simulink model "ps_25V_12kA_r"  (R2026b)
settings: Solver=ode23tb  StopTime=param.sim.simlength  FixedStep=param.glb_time.tc  MaxStep=param.glb_time.tc
values from neighbouring files (symbols this model uses):
  param = struct()    [init_model.m]
undefined symbols (not defined in the file or in its folder): magnitude
libraries: fl_lib x106, nesl_utility x71, afe_uvw_ctrl x5, ee_legacy_lib x5, discrete_time_low_pass_filter x2, three_windings_transformer x2, pi_ctrl x2, threephase_inductor_lib x1, dclink_for_two_levels x1, three_phase_pwm_modulator x1, three_phase_inverter_ideal_switch_based_model x1, three_phase_inverter_igbt_advanced_thermal_model x1
(part 1 of 5)
settings Model: Creator=dbagn  LastModifiedBy=d.bagnara
settings SolverCC: SolverResetMethod=Robust  ZeroCrossControl=DisableAll
settings DataIOCC: DSMLogging=off  ReturnWorkspaceOutputs=off  SaveOutput=off  SaveTime=off  SignalLogging=off
settings OptimizationCC: ReuseModelBlockBuffer=off
settings SFSimCC: CustomCodeUndefinedFunction=ThrowError  DefaultCustomCodeDeterministicFunctions=All
settings SFSimCC: SimCustomHeaderCode=|
  | #include "rpi.h"
  | #include "mavgflt.h"
  | #include "mavgflt_simulink.h"
  | #include "mavgflts.h"
  | #include "mavgflts_simulink.h"
  | #include "dsmavgflt.h"
  | #include "dsmavgflt_simulink.h"
  | #include "bemf_obsv.h"
  | #include "bemf_obsv_simulink.h"
  | #include "bemf_obsv_load_est.h"
  | #include "bemf_obsv_load_est_simulink.h"
  | #include "dqvector_pi.h"
  | #include "dqvector_pi_simulink.h"
  | #include "sv_pwm_simulink.h"
  | #include "sv_pwm.h"
  | #include "sv_pwm_cm_simulink.h"
  | #include "sv_pwm_cm.h"
  | #include "first_harmonic_tracker.h"
  | #include "first_harmonic_tracker_simulink.h"
  | #include "dqpll_thyr.h"
  | #include "dqpll_thyr_simulink.h"
  | #include "dqpll_grid.h"
  | #include "dqpll_grid_simulink.h"
  | #include "linear_double_integrator_observer_simulink.h"
  | #include "linear_double_integrator_observer.h"
settings SFSimCC: SimUserIncludeDirs=|
  | include
  | src
settings SFSimCC: SimUserSources=|
  | "rpi.c"
  | "mavgflt_simulink.c"
  | "mavgflt.c"
  | "mavgflts_simulink.c"
  | "mavgflts.c"
  | "dsmavgflt_simulink.c"
  | "dsmavgflt.c"
  | "bemf_obsv_simulink.c"
  | "bemf_obsv.c"
  | "bemf_obsv_load_est_simulink.c"
  | "bemf_obsv_load_est.c"
  | "dqvector_pi.c"
  | "dqvector_pi_simulink.c"
  | "sv_pwm_simulink.c"
  | "sv_pwm.c"
  | "sv_pwm_cm_simulink.c"
  | "sv_pwm_cm.c"
  | "first_harmonic_tracker_simulink.c"
  | "first_harmonic_tracker.c"
  | "dqpll_thyr_simulink.c"
  | "dqpll_thyr.c"
  | "dqpll_grid_simulink.c"
  | "dqpll_grid.c"
  | "linear_double_integrator_observer_simulink.c"
  | "linear_double_integrator_observer.c"
settings RTWCC: DLArmComputeVersion=19.05
settings SimscapeCC: SimscapeUseEnergyAccounting=off

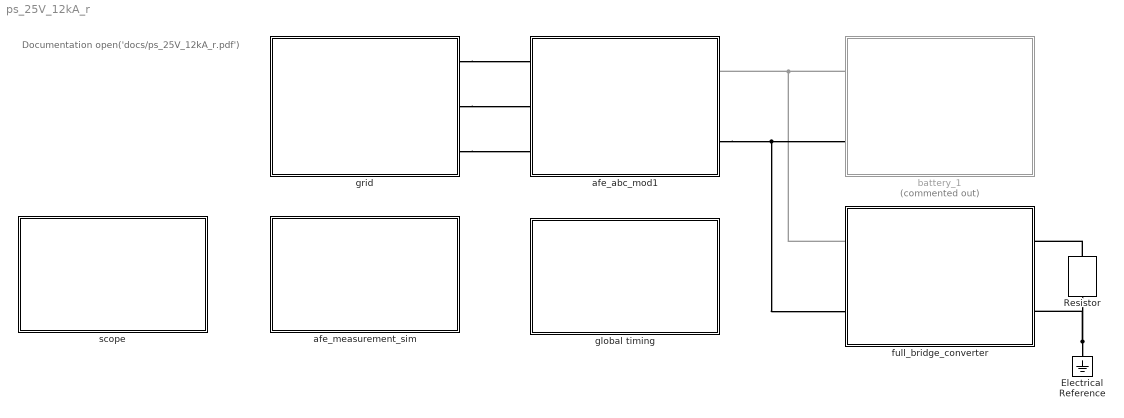
== system ps_25V_12kA_r ==
  note: Documentation
      | open('docs/ps_25V_12kA_r.pdf')
  Electrical Reference : fl_lib/Electrical/Electrical Elements/Electrical Reference
  Resistor : fl_lib/Electrical/Electrical Elements/Resistor  R=param.load.R Ohm  i_specify=off  i_priority=None  i=0 A  i_nominal_specify=off  i_nominal_value=1  i_nominal_unit=A  v_specify=off  v_priority=None  v=0 V  v_nominal_specify=off  v_nominal_value=1  v_nominal_unit=V
  afe_abc_mod1 : Subsystem
  afe_measurement_sim : Subsystem
  battery_1 : Subsystem  Commented=on
  full_bridge_converter : Subsystem
  global timing : Subsystem
  grid : Subsystem
  scope : Subsystem
  connections:
  grid/RConn1 -- afe_abc_mod1/LConn1
  grid/RConn3 -- afe_abc_mod1/LConn3
  grid/RConn2 -- afe_abc_mod1/LConn2
  battery_1/RConn1 -- full_bridge_converter/LConn1 -- afe_abc_mod1/RConn1
  afe_abc_mod1/RConn2 -- full_bridge_converter/LConn2 -- battery_1/RConn2
  Electrical Reference/LConn1 -- Resistor/RConn1 -- full_bridge_converter/RConn2
  Resistor/LConn1 -- full_bridge_converter/RConn1

== system ps_25V_12kA_r/afe_abc_mod1 ==
  AFE_control : Subsystem
  LCL_filter : Subsystem
  afe : Subsystem
  brake : Subsystem
  ug_a : PMIOPort  Side=Left
  Udc(+) : PMIOPort  Port=2  Side=Right
  ug_b : PMIOPort  Port=3  Side=Left
  Udc(-) : PMIOPort  Port=4  Side=Right
  ug_c : PMIOPort  Port=5  Side=Left
  wires:
  AFE_control/1(dabc_out) -> afe/1(dabc)
  connections:
  Udc(-)/RConn1 -- brake/LConn2 -- afe/RConn2
  Udc(+)/RConn1 -- brake/LConn1 -- afe/RConn1
  LCL_filter/LConn1 -- afe/LConn1
  LCL_filter/LConn2 -- afe/LConn2
  LCL_filter/LConn3 -- afe/LConn3
  ug_a/RConn1 -- LCL_filter/RConn1
  ug_b/RConn1 -- LCL_filter/RConn2
  ug_c/RConn1 -- LCL_filter/RConn3

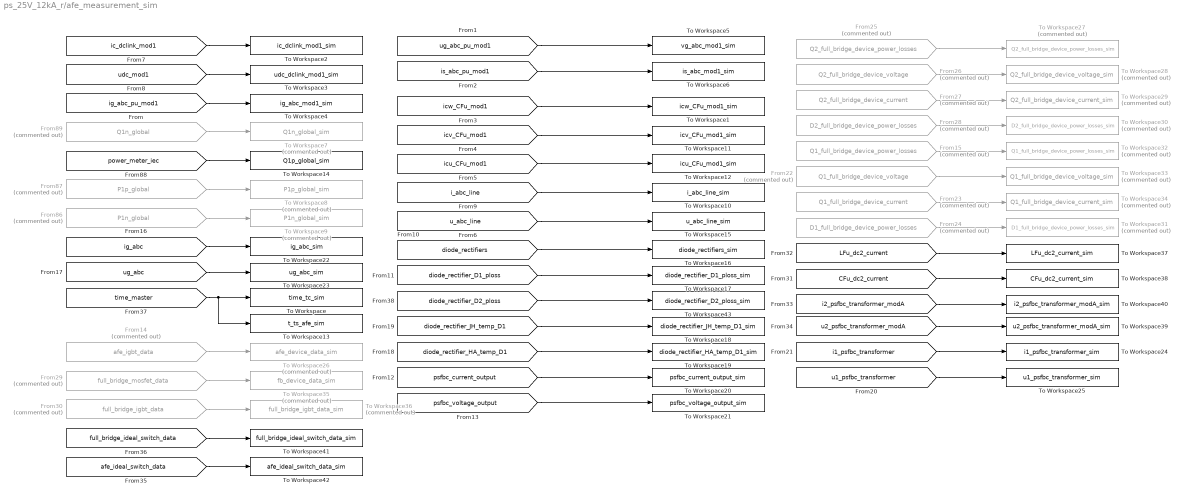
== system ps_25V_12kA_r/afe_measurement_sim ==
  From14 : From  Commented=on  GotoTag=afe_igbt_data
  From15 : From  Commented=on  GotoTag=Q1_full_bridge_device_power_losses
  From22 : From  Commented=on  GotoTag=Q1_full_bridge_device_voltage
  From23 : From  Commented=on  GotoTag=Q1_full_bridge_device_current
  From24 : From  Commented=on  GotoTag=D1_full_bridge_device_power_losses
  From25 : From  Commented=on  GotoTag=Q2_full_bridge_device_power_losses
  From26 : From  Commented=on  GotoTag=Q2_full_bridge_device_voltage
  From27 : From  Commented=on  GotoTag=Q2_full_bridge_device_current
  From28 : From  Commented=on  GotoTag=D2_full_bridge_device_power_losses
  From29 : From  Commented=on  GotoTag=full_bridge_mosfet_data
  From30 : From  Commented=on  GotoTag=full_bridge_igbt_data
  From86 : From  Commented=on  GotoTag=P1n_global
  From87 : From  Commented=on  GotoTag=P1p_global
  From89 : From  Commented=on  GotoTag=Q1n_global
  To Workspace : ToWorkspace  VariableName=time_tc_sim  SampleTime=param.glb_time.tc
      settings: MaxDataPoints=param.glb_time.Nc  Decimation=param.glb_time.decimation_tc
  To Workspace1 : ToWorkspace  VariableName=icw_CFu_mod1_sim  SampleTime=param.glb_time.tc
      settings: MaxDataPoints=param.glb_time.Nc  Decimation=param.glb_time.decimation_tc
  To Workspace10 : ToWorkspace  VariableName=i_abc_line_sim  SampleTime=param.glb_time.tc
      settings: MaxDataPoints=param.glb_time.Nc  Decimation=param.glb_time.decimation_tc
  To Workspace11 : ToWorkspace  VariableName=icv_CFu_mod1_sim  SampleTime=param.glb_time.tc
      settings: MaxDataPoints=param.glb_time.Nc  Decimation=param.glb_time.decimation_tc
  To Workspace12 : ToWorkspace  VariableName=icu_CFu_mod1_sim  SampleTime=param.glb_time.tc
      settings: MaxDataPoints=param.glb_time.Nc  Decimation=param.glb_time.decimation_tc
  To Workspace13 : ToWorkspace  VariableName=t_ts_afe_sim  SampleTime=param.glb_time.ts_afe
      settings: MaxDataPoints=param.glb_time.Ns_afe
  To Workspace14 : ToWorkspace  VariableName=Q1p_global_sim  SampleTime=param.glb_time.tc
      settings: MaxDataPoints=param.glb_time.Nc  Decimation=param.glb_time.decimation_tc
  To Workspace15 : ToWorkspace  VariableName=u_abc_line_sim  SampleTime=param.glb_time.tc
      settings: MaxDataPoints=param.glb_time.Nc  Decimation=param.glb_time.decimation_tc
  To Workspace16 : ToWorkspace  VariableName=diode_rectifiers_sim  SampleTime=param.glb_time.tc
      settings: MaxDataPoints=param.glb_time.Nc  Decimation=param.glb_time.decimation_tc
  To Workspace17 : ToWorkspace  VariableName=diode_rectifier_D1_ploss_sim  SampleTime=param.glb_time.tc
      settings: MaxDataPoints=param.glb_time.Nc  Decimation=param.glb_time.decimation_tc
  To Workspace18 : ToWorkspace  VariableName=diode_rectifier_JH_temp_D1_sim  SampleTime=param.glb_time.tc
      settings: MaxDataPoints=param.glb_time.Nc  Decimation=param.glb_time.decimation_tc
  To Workspace19 : ToWorkspace  VariableName=diode_rectifier_HA_temp_D1_sim  SampleTime=param.glb_time.tc
      settings: MaxDataPoints=param.glb_time.Nc  Decimation=param.glb_time.decimation_tc
  To Workspace2 : ToWorkspace  VariableName=ic_dclink_mod1_sim  SampleTime=param.glb_time.tc
      settings: MaxDataPoints=param.glb_time.Nc  Decimation=param.glb_time.decimation_tc
  To Workspace20 : ToWorkspace  VariableName=psfbc_current_output_sim  SampleTime=param.glb_time.tc
      settings: MaxDataPoints=param.glb_time.Nc  Decimation=param.glb_time.decimation_tc
  To Workspace21 : ToWorkspace  VariableName=psfbc_voltage_output_sim  SampleTime=param.glb_time.tc
      settings: MaxDataPoints=param.glb_time.Nc  Decimation=param.glb_time.decimation_tc
  To Workspace22 : ToWorkspace  VariableName=ig_abc_sim  SampleTime=param.glb_time.tc
      settings: MaxDataPoints=param.glb_time.Nc  Decimation=param.glb_time.decimation_tc
  To Workspace23 : ToWorkspace  VariableName=ug_abc_sim  SampleTime=param.glb_time.tc
      settings: MaxDataPoints=param.glb_time.Nc  Decimation=param.glb_time.decimation_tc
  To Workspace24 : ToWorkspace  VariableName=i1_psfbc_transformer_sim  SampleTime=param.glb_time.tc
      settings: MaxDataPoints=param.glb_time.Nc  Decimation=param.glb_time.decimation_tc
  To Workspace25 : ToWorkspace  VariableName=u1_psfbc_transformer_sim  SampleTime=param.glb_time.tc
      settings: MaxDataPoints=param.glb_time.Nc  Decimation=param.glb_time.decimation_tc
  To Workspace26 : ToWorkspace  Commented=on  VariableName=afe_device_data_sim  SampleTime=param.glb_time.tc
      settings: MaxDataPoints=param.glb_time.Nc  Decimation=param.glb_time.decimation_tc
  To Workspace27 : ToWorkspace  Commented=on  VariableName=Q2_full_bridge_device_power_losses_sim  SampleTime=param.glb_time.tc
      settings: MaxDataPoints=param.glb_time.Nc  Decimation=param.glb_time.decimation_tc
  To Workspace28 : ToWorkspace  Commented=on  VariableName=Q2_full_bridge_device_voltage_sim  SampleTime=param.glb_time.tc
      settings: MaxDataPoints=param.glb_time.Nc  Decimation=param.glb_time.decimation_tc
  To Workspace29 : ToWorkspace  Commented=on  VariableName=Q2_full_bridge_device_current_sim  SampleTime=param.glb_time.tc
      settings: MaxDataPoints=param.glb_time.Nc  Decimation=param.glb_time.decimation_tc
  To Workspace3 : ToWorkspace  VariableName=udc_dclink_mod1_sim  SampleTime=param.glb_time.tc
      settings: MaxDataPoints=param.glb_time.Nc  Decimation=param.glb_time.decimation_tc
  To Workspace30 : ToWorkspace  Commented=on  VariableName=D2_full_bridge_device_power_losses_sim  SampleTime=param.glb_time.tc
      settings: MaxDataPoints=param.glb_time.Nc  Decimation=param.glb_time.decimation_tc
  To Workspace31 : ToWorkspace  Commented=on  VariableName=D1_full_bridge_device_power_losses_sim  SampleTime=param.glb_time.tc
      settings: MaxDataPoints=param.glb_time.Nc  Decimation=param.glb_time.decimation_tc
  To Workspace32 : ToWorkspace  Commented=on  VariableName=Q1_full_bridge_device_power_losses_sim  SampleTime=param.glb_time.tc
      settings: MaxDataPoints=param.glb_time.Nc  Decimation=param.glb_time.decimation_tc
  To Workspace33 : ToWorkspace  Commented=on  VariableName=Q1_full_bridge_device_voltage_sim  SampleTime=param.glb_time.tc
      settings: MaxDataPoints=param.glb_time.Nc  Decimation=param.glb_time.decimation_tc
  To Workspace34 : ToWorkspace  Commented=on  VariableName=Q1_full_bridge_device_current_sim  SampleTime=param.glb_time.tc
      settings: MaxDataPoints=param.glb_time.Nc  Decimation=param.glb_time.decimation_tc
  To Workspace35 : ToWorkspace  Commented=on  VariableName=fb_device_data_sim  SampleTime=param.glb_time.tc
      settings: MaxDataPoints=param.glb_time.Nc  Decimation=param.glb_time.decimation_tc
  To Workspace36 : ToWorkspace  Commented=on  VariableName=full_bridge_igbt_data_sim  SampleTime=param.glb_time.tc
      settings: MaxDataPoints=param.glb_time.Nc  Decimation=param.glb_time.decimation_tc
  To Workspace37 : ToWorkspace  VariableName=LFu_dc2_current_sim  SampleTime=param.glb_time.tc
      settings: MaxDataPoints=param.glb_time.Nc  Decimation=param.glb_time.decimation_tc
  To Workspace38 : ToWorkspace  VariableName=CFu_dc2_current_sim  SampleTime=param.glb_time.tc
      settings: MaxDataPoints=param.glb_time.Nc  Decimation=param.glb_time.decimation_tc
  To Workspace39 : ToWorkspace  VariableName=u2_psfbc_transformer_modA_sim  SampleTime=param.glb_time.tc
      settings: MaxDataPoints=param.glb_time.Nc  Decimation=param.glb_time.decimation_tc
  To Workspace4 : ToWorkspace  VariableName=ig_abc_mod1_sim  SampleTime=param.glb_time.tc
      settings: MaxDataPoints=param.glb_time.Nc  Decimation=param.glb_time.decimation_tc
  To Workspace40 : ToWorkspace  VariableName=i2_psfbc_transformer_modA_sim  SampleTime=param.glb_time.tc
      settings: MaxDataPoints=param.glb_time.Nc  Decimation=param.glb_time.decimation_tc
  To Workspace41 : ToWorkspace  VariableName=full_bridge_ideal_switch_data_sim  SampleTime=param.glb_time.tc
      settings: MaxDataPoints=param.glb_time.Nc  Decimation=param.glb_time.decimation_tc
  To Workspace42 : ToWorkspace  VariableName=afe_ideal_switch_data_sim  SampleTime=param.glb_time.tc
      settings: MaxDataPoints=param.glb_time.Nc  Decimation=param.glb_time.decimation_tc
  To Workspace43 : ToWorkspace  VariableName=diode_rectifier_D2_ploss_sim  SampleTime=param.glb_time.tc
      settings: MaxDataPoints=param.glb_time.Nc  Decimation=param.glb_time.decimation_tc
  To Workspace5 : ToWorkspace  VariableName=vg_abc_mod1_sim  SampleTime=param.glb_time.tc
      settings: MaxDataPoints=param.glb_time.Nc  Decimation=param.glb_time.decimation_tc
  To Workspace6 : ToWorkspace  VariableName=is_abc_mod1_sim  SampleTime=param.glb_time.tc
      settings: MaxDataPoints=param.glb_time.Nc  Decimation=param.glb_time.decimation_tc
  To Workspace7 : ToWorkspace  Commented=on  VariableName=Q1n_global_sim  SampleTime=param.glb_time.tc
      settings: MaxDataPoints=param.glb_time.Nc  Decimation=param.glb_time.decimation_tc
  To Workspace8 : ToWorkspace  Commented=on  VariableName=P1p_global_sim  SampleTime=param.glb_time.tc
      settings: MaxDataPoints=param.glb_time.Nc  Decimation=param.glb_time.decimation_tc
  To Workspace9 : ToWorkspace  Commented=on  VariableName=P1n_global_sim  SampleTime=param.glb_time.tc
      settings: MaxDataPoints=param.glb_time.Nc  Decimation=param.glb_time.decimation_tc
  wires:
  [time_master] -> To Workspace13/1, To Workspace/1
  From89/1 -> To Workspace7/1
  [power_meter_iec] -> To Workspace14/1
  From87/1 -> To Workspace8/1
  From86/1 -> To Workspace9/1
  [ug_abc] -> To Workspace23/1
  [ig_abc] -> To Workspace22/1
  [ug_abc_pu_mod1] -> To Workspace5/1
  [ig_abc_pu_mod1] -> To Workspace4/1
  [udc_mod1] -> To Workspace3/1
  [ic_dclink_mod1] -> To Workspace2/1
  [is_abc_pu_mod1] -> To Workspace6/1
  [icw_CFu_mod1] -> To Workspace1/1
  [icv_CFu_mod1] -> To Workspace11/1
  [icu_CFu_mod1] -> To Workspace12/1
  [i_abc_line] -> To Workspace10/1
  [u_abc_line] -> To Workspace15/1
  [diode_rectifiers] -> To Workspace16/1
  [diode_rectifier_JH_temp_D1] -> To Workspace18/1
  [diode_rectifier_D1_ploss] -> To Workspace17/1
  [diode_rectifier_HA_temp_D1] -> To Workspace19/1
  [psfbc_current_output] -> To Workspace20/1
  [psfbc_voltage_output] -> To Workspace21/1
  [i1_psfbc_transformer] -> To Workspace24/1
  [u1_psfbc_transformer] -> To Workspace25/1
  From14/1 -> To Workspace26/1
  From25/1 -> To Workspace27/1
  From26/1 -> To Workspace28/1
  From27/1 -> To Workspace29/1
  From15/1 -> To Workspace32/1
  From22/1 -> To Workspace33/1
  From23/1 -> To Workspace34/1
  From28/1 -> To Workspace30/1
  From24/1 -> To Workspace31/1
  From29/1 -> To Workspace35/1
  From30/1 -> To Workspace36/1
  [LFu_dc2_current] -> To Workspace37/1
  [CFu_dc2_current] -> To Workspace38/1
  [u2_psfbc_transformer_modA] -> To Workspace39/1
  [i2_psfbc_transformer_modA] -> To Workspace40/1
  [full_bridge_ideal_switch_data] -> To Workspace41/1
  [afe_ideal_switch_data] -> To Workspace42/1
  [diode_rectifier_D2_ploss] -> To Workspace43/1

== system ps_25V_12kA_r/battery_1 ==
  Electrical Reference : fl_lib/Electrical/Electrical Elements/Electrical Reference
  Inductor : fl_lib/Electrical/Electrical Elements/Inductor  l=1e-3 H  r=0 Ohm  g=1e-9 1/Ohm  i_specify=off  i_priority=None  i=0 A  i_nominal_specify=off  i_nominal_value=1  i_nominal_unit=A  v_specify=off  v_priority=None  v=0 V  v_nominal_specify=off  v_nominal_value=1  v_nominal_unit=V  i_L_specify=off  i_L_priority=High  i_L=0 A  i_L_nominal_specify=off  i_L_nominal_value=1  i_L_nominal_unit=A
  Solver Configuration : nesl_utility/Solver Configuration  PhysicalDomain=network_engine_domain  SubClassName=solver  LeftPortType=input  RightPortType=generic  Tones=[]  Harmonics=[]  SimulateNoise=off  Profile=off  UseLocalSampling=off  EnableSwitchedLinearOptims=on  FrequencyDomain=off  UseCCode=off  RelTol=0.001  AbsTol=0.001  MinStep=1e-09  ToWorkspace=off  RevertToSquareIcSolve=off  NumHomotopyIterations=100  PhasorMode=off  PhasorModeNumHarmonics=1  ConsistencySolver=NEWTON_FTOL  CanonicalOrdering=UNORDERED  OptimizeIntermediates=UNOPTIMIZED  MulticoreSolverChoice=BACKWARD_EULER  IndexReductionMethod=DerivativeReplacement  DoDC=on  ResidualTolerance=1e-3  ConsistencyTolSource=GLOBAL  ConsistencyAbsTol=0.001  ConsistencyRelTol=0.001  ConsistencyTolFactor=0.001  UseLocalSolver=on  LocalSolverChoice=NE_BACKWARD_EULER_ADVANCER  ResolveIndetEquations=on  FunctionEvalNumThread=1  LocalSolverSampleTime=param.glb_time.tc  DoFixedCost=on  MaxNonlinIter=param.sim.nonlinear_iterations  MaxModeIter=2  ComputeImpulses=off  ImpulseIterations=2  LinearAlgebra=auto  LinearAlgebraNumThread=0  EquationFormulation=NE_TIME_EF  DelaysMemoryBudget=1024  AutomaticFiltering=on  FilteringTimeConstant=0.001  PartitionStorageMethod=AS_NEEDED  PartitionMemoryBudget=1024  PartitionMethod=BALANCED  MultibodyUseLocalSolver=off  MultibodyLocalSolverChoice=ODE1  MultibodyLocalSolverSampleTime=0.001
  To Workspace14 : ToWorkspace  VariableName=battery_1_data_sim  SampleTime=param.glb_time.tc
      settings: MaxDataPoints=param.glb_time.Nc  Decimation=param.glb_time.decimation_tc
  lithium ion battery : Scope
      settings: ActiveDisplayYMinimum=-808.27997881012811  ActiveDisplayYMaximum=1287.7546757937268  DataLoggingVariableName=ScopeData3
  lithium_ion_battery : lithium_ion_battery/lithium_ion_battery  Q=param.battery.pack_1.Q  number_of_cells=param.battery.pack_1.number_of_cells  E_1=param.battery.pack_1.E_1  E0=param.battery.pack_1.E0  E1=param.battery.pack_1.E1  E2=param.battery.pack_1.E2  E3=param.battery.pack_1.E3  Elog=param.battery.pack_1.Elog  R0=param.battery.pack_1.R0  R1=param.battery.pack_1.R1  C1=param.battery.pack_1.C1  M=param.battery.pack_1.M  alpha=param.battery.pack_1.alpha  soc_init=param.battery.pack_1.soc_init  ts_battery=param.glb_time.ts_dab  q1Kalman=param.battery.pack_1.q1Kalman  q2Kalman=param.battery.pack_1.q2Kalman  q3Kalman=param.battery.pack_1.q3Kalman  rKalman=param.battery.pack_1.rKalman  tc=param.glb_time.tc  enable_white_noise_m=0  battery_voltage_init_m=param.battery.nominal_battery_voltage_1
  single_phase_ui_measure : Subsystem
  dc(+) : PMIOPort  Side=Right
  dc(-) : PMIOPort  Port=2  Side=Right
  wires:
  lithium_ion_battery/1 -> To Workspace14/1, lithium ion battery/1
  connections:
  Solver Configuration/RConn1 -- lithium_ion_battery/RConn2 -- single_phase_ui_measure/LConn2 -- Electrical Reference/LConn1
  single_phase_ui_measure/RConn1 -- dc(+)/RConn1
  Inductor/LConn1 -- lithium_ion_battery/RConn1
  dc(-)/RConn1 -- single_phase_ui_measure/RConn2
  single_phase_ui_measure/LConn1 -- Inductor/RConn1

== system ps_25V_12kA_r/full_bridge_converter ==
  full_bridge_converter_with_iso : Subsystem
  phase_shift_full_bridge_ctrl : Subsystem
  udc(+) : PMIOPort  Side=Right
  udc(-) : PMIOPort  Port=2  Side=Right
  dc+ : PMIOPort  Port=3  Side=Left
  dc- : PMIOPort  Port=4  Side=Left
  wires:
  phase_shift_full_bridge_ctrl/1(gate_cmds) -> full_bridge_converter_with_iso/1(gate_cmds)
  connections:
  udc(+)/RConn1 -- full_bridge_converter_with_iso/RConn1
  udc(-)/RConn1 -- full_bridge_converter_with_iso/RConn2
  dc-/RConn1 -- full_bridge_converter_with_iso/LConn2
  dc+/RConn1 -- full_bridge_converter_with_iso/LConn1

== system ps_25V_12kA_r/global timing ==
  Unit Delay : UnitDelay  SampleTime=param.glb_time.tc
  Unit Delay4 : UnitDelay  SampleTime=param.glb_time.tc
  pwm_alignments : Scope
      settings: SampleTime=param.glb_time.tc  ActiveDisplayYMinimum=-0.0023956891982955782  ActiveDisplayYMaximum=0.0016011229443397596  DataLoggingVariableName=ScopeData40
  time_afe1 : Subsystem  mask{k=param.afe.behav.time_gain_module_1}
      mask prompts: k "Time Gain"
      mask Display:
      | disp('time-gen');
      | port_label('input', 1, 'crt');
      | port_label('output', 1, 'tout');
  time_fbc1 : Subsystem  mask{k=1}
      mask prompts: k "Time Gain"
      mask Display:
      | disp('time-gen');
      | port_label('input', 1, 'crt');
      | port_label('output', 1, 'tout');
  time_master : Subsystem  mask{k=1}
      mask prompts: k "Time Gain"
      mask Display:
      | disp('time-gen');
      | port_label('output', 1, 'tout');
  tag scope: time_afe_module_1=global, time_master=global, time_psfbc_module_1=global
  wires:
  time_afe1/1(Out1) -> [time_afe_module_1]
  time_master/1(Out1) -> [time_master]
  Unit Delay/1 -> time_afe1/1(correction_time)
  [local_time_corr_afe1] -> pwm_alignments/1  "local_time_corr_afe1"
  [local_time_corr_afe1] -> Unit Delay/1
  Unit Delay4/1 -> time_fbc1/1(correction_time)
  time_fbc1/1(Out1) -> [time_psfbc_module_1]

== system ps_25V_12kA_r/grid ==
  grid_emulator : Subsystem
  power meter iec mfunc : Subsystem
  threephase_vi_measures : Subsystem
  ua : PMIOPort  Side=Right
  ub : PMIOPort  Port=2  Side=Right
  uc : PMIOPort  Port=3  Side=Right
  connections:
  threephase_vi_measures/LConn3 -- grid_emulator/RConn3
  threephase_vi_measures/LConn1 -- grid_emulator/RConn1
  threephase_vi_measures/RConn2 -- ub/RConn1
  threephase_vi_measures/LConn2 -- grid_emulator/RConn2
  threephase_vi_measures/RConn1 -- ua/RConn1
  threephase_vi_measures/RConn3 -- uc/RConn1

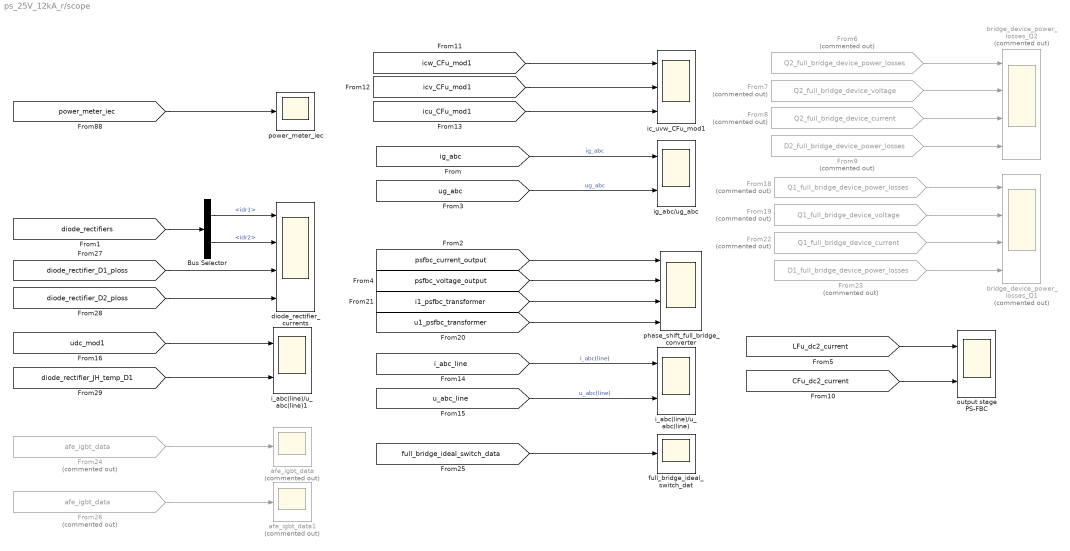
== system ps_25V_12kA_r/scope ==
  Bus Selector : BusSelector  OutputSignals=idr1,idr2
  From18 : From  Commented=on  GotoTag=Q1_full_bridge_device_power_losses
  From19 : From  Commented=on  GotoTag=Q1_full_bridge_device_voltage
  From22 : From  Commented=on  GotoTag=Q1_full_bridge_device_current
  From23 : From  Commented=on  GotoTag=D1_full_bridge_device_power_losses
  From24 : From  Commented=on  GotoTag=afe_igbt_data
  From26 : From  Commented=on  GotoTag=afe_igbt_data
  From6 : From  Commented=on  GotoTag=Q2_full_bridge_device_power_losses
  From7 : From  Commented=on  GotoTag=Q2_full_bridge_device_voltage
  From8 : From  Commented=on  GotoTag=Q2_full_bridge_device_current
  From9 : From  Commented=on  GotoTag=D2_full_bridge_device_power_losses
  afe_igbt_data : Scope  Commented=on
      settings: SampleTime=param.glb_time.tc  ActiveDisplayYMinimum=-185.80082711442992  ActiveDisplayYMaximum=1530.3864871069391  DataLoggingVariableName=ScopeData24
  afe_igbt_data1 : Scope  Commented=on
      settings: SampleTime=param.glb_time.tc  ActiveDisplayYMinimum=-185.80082711442992  ActiveDisplayYMaximum=1530.3864871069391  DataLoggingVariableName=ScopeData26
  bridge_device_power_losses_Q1 : Scope  Commented=on  NumInputPorts=4
      settings: SampleTime=param.glb_time.tc  ActiveDisplayYMinimum=-132.81353179927618  ActiveDisplayYMaximum=1178.2847224343986  DataLoggingVariableName=ScopeData23
  bridge_device_power_losses_Q2 : Scope  Commented=on  NumInputPorts=4
      settings: SampleTime=param.glb_time.tc  ActiveDisplayYMinimum=-102.91748468374873  ActiveDisplayYMaximum=909.22247743852836  DataLoggingVariableName=ScopeData20
  diode_rectifier_currents : Scope  NumInputPorts=4
      settings: ActiveDisplayString=3  ActiveDisplayYMinimum=-723.410067277231  ActiveDisplayYMaximum=6510.6902367425982  DataLoggingVariableName=ScopeData11
  full_bridge_ideal_switch_dat : Scope
      settings: SampleTime=param.glb_time.tc  ActiveDisplayYMinimum=-185.80082711442992  ActiveDisplayYMaximum=1530.3864871069391  DataLoggingVariableName=ScopeData25
  i_abc(line)/u_abc(line) : Scope  NumInputPorts=2
      settings: SampleTime=param.glb_time.tc  ActiveDisplayYMinimum=-489.89793495771346  ActiveDisplayYMaximum=489.89793495771346  DataLoggingVariableName=ScopeData18
  i_abc(line)/u_abc(line)1 : Scope  NumInputPorts=2
      settings: SampleTime=param.glb_time.tc  ActiveDisplayYMinimum=-1  ActiveDisplayYMaximum=1  DataLoggingVariableName=ScopeData19
  ic_uvw_CFu_mod1 : Scope  NumInputPorts=3
      settings: SampleTime=param.glb_time.tc  ActiveDisplayYMinimum=-250.78571798939993  ActiveDisplayYMaximum=408.17461480787006  DataLoggingVariableName=ScopeData17
  ig_abc/ug_abc : Scope  NumInputPorts=2
      settings: SampleTime=param.glb_time.tc  ActiveDisplayYMinimum=-494.737319512461  ActiveDisplayYMaximum=494.80225542196177  DataLoggingVariableName=ScopeData15
  output stage PS-FBC : Scope  NumInputPorts=2
      settings: SampleTime=param.glb_time.tc  ActiveDisplayYMinimum=-658.65362756432182  ActiveDisplayYMaximum=664.76716339933853  DataLoggingVariableName=ScopeData22
  phase_shift_full_bridge_converter : Scope  NumInputPorts=4
      settings: SampleTime=param.glb_time.tc  ActiveDisplayYMinimum=-1597.686541193829  ActiveDisplayYMaximum=14379.178870744465  DataLoggingVariableName=ScopeData16
  power_meter_iec : Scope
      settings: SampleTime=param.glb_time.tc  ActiveDisplayYMinimum=-185.80082711442992  ActiveDisplayYMaximum=1530.3864871069391  DataLoggingVariableName=ScopeData27
  wires:
  [ug_abc] -> ig_abc/ug_abc/2  "ug_abc"
  [ig_abc] -> ig_abc/ug_abc/1  "ig_abc"
  [icw_CFu_mod1] -> ic_uvw_CFu_mod1/1
  [icv_CFu_mod1] -> ic_uvw_CFu_mod1/2
  [icu_CFu_mod1] -> ic_uvw_CFu_mod1/3
  [i_abc_line] -> i_abc(line)/u_abc(line)/1  "i_abc(line)"
  [u_abc_line] -> i_abc(line)/u_abc(line)/2  "u_abc(line)"
  [udc_mod1] -> i_abc(line)/u_abc(line)1/1
  [diode_rectifiers] -> Bus Selector/1
  [psfbc_current_output] -> phase_shift_full_bridge_converter/1
  [psfbc_voltage_output] -> phase_shift_full_bridge_converter/2
  [i1_psfbc_transformer] -> phase_shift_full_bridge_converter/3
  [u1_psfbc_transformer] -> phase_shift_full_bridge_converter/4
  Bus Selector/1 -> diode_rectifier_currents/1  "<idr1>"
  Bus Selector/2 -> diode_rectifier_currents/2  "<idr2>"
  [LFu_dc2_current] -> output stage PS-FBC/1
  [CFu_dc2_current] -> output stage PS-FBC/2
  From6/1 -> bridge_device_power_losses_Q2/1
  From7/1 -> bridge_device_power_losses_Q2/2
  From8/1 -> bridge_device_power_losses_Q2/3
  From9/1 -> bridge_device_power_losses_Q2/4
  From18/1 -> bridge_device_power_losses_Q1/1
  From19/1 -> bridge_device_power_losses_Q1/2
  From22/1 -> bridge_device_power_losses_Q1/3
  From23/1 -> bridge_device_power_losses_Q1/4
  From24/1 -> afe_igbt_data/1
  [full_bridge_ideal_switch_data] -> full_bridge_ideal_switch_dat/1
  From26/1 -> afe_igbt_data1/1
  [diode_rectifier_D1_ploss] -> diode_rectifier_currents/3
  [diode_rectifier_D2_ploss] -> diode_rectifier_currents/4
  [diode_rectifier_JH_temp_D1] -> i_abc(line)/u_abc(line)1/2
  [power_meter_iec] -> power_meter_iec/1

== system ps_25V_12kA_r/afe_abc_mod1/AFE_control ==
  To Workspace : ToWorkspace  VariableName=afe_ctrl_data_output_mod1  SampleTime=param.glb_time.ts_afe
      settings: MaxDataPoints=param.glb_time.Ns_afe
  afe_control : Subsystem
  dabc_out : Outport
  tag scope: local_time_corr_afe1=global
  wires:
  [TRGO_afe_module_1] -> afe_control/Trigger
  [ug_abc_pu_mod1] -> afe_control/1(ug_abc_pu)
  [is_abc_pu_mod1] -> afe_control/4(is_abc_pu)
  [vdc_pu_afe_mod1] -> afe_control/2(udc_pu)
  afe_control/1(duvw) -> dabc_out/1
  [ig_abc_pu_mod1] -> afe_control/3(ig_abc_pu)
  [time_afe_module_1] -> afe_control/5(local_time)
  [time_master] -> afe_control/6(master_time)
  [phase_grid_emulator] -> afe_control/7(grid_phase)
  afe_control/3(m_data) -> To Workspace/1
  afe_control/2(AFE1_local_time_corr) -> [local_time_corr_afe1]

== system ps_25V_12kA_r/afe_abc_mod1/LCL_filter ==
  CapacitorFilter : Subsystem
  Inductor : fl_lib/Electrical/Electrical Elements/Inductor  l=1e-6 H  r=0 Ohm  g=1e-9 1/Ohm  i_specify=on  i_priority=High  i=0 A  i_nominal_specify=off  i_nominal_value=1  i_nominal_unit=A  v_specify=off  v_priority=None  v=0 V  v_nominal_specify=off  v_nominal_value=1  v_nominal_unit=V  i_L_specify=off  i_L_priority=High  i_L=0 A  i_L_nominal_specify=off  i_L_nominal_value=1  i_L_nominal_unit=A
  Inductor1 : fl_lib/Electrical/Electrical Elements/Inductor  l=1e-6 H  r=0 Ohm  g=1e-9 1/Ohm  i_specify=on  i_priority=High  i=0 A  i_nominal_specify=off  i_nominal_value=1  i_nominal_unit=A  v_specify=off  v_priority=None  v=0 V  v_nominal_specify=off  v_nominal_value=1  v_nominal_unit=V  i_L_specify=off  i_L_priority=High  i_L=0 A  i_L_nominal_specify=off  i_L_nominal_value=1  i_L_nominal_unit=A
  Inductor2 : fl_lib/Electrical/Electrical Elements/Inductor  l=1e-6 H  r=0 Ohm  g=1e-9 1/Ohm  i_specify=on  i_priority=High  i=0 A  i_nominal_specify=off  i_nominal_value=1  i_nominal_unit=A  v_specify=off  v_priority=None  v=0 V  v_nominal_specify=off  v_nominal_value=1  v_nominal_unit=V  i_L_specify=off  i_L_priority=High  i_L=0 A  i_L_nominal_specify=off  i_L_nominal_value=1  i_L_nominal_unit=A
  threephase inductor : threephase_inductor_lib/threephase inductor  Lp=param.afe.hw.LFu H  L0=param.afe.hw.LFu_cm H  Rp=param.afe.hw.RLFu Ohm  R0=param.afe.hw.RLFu_cm Ohm  Lls=5e-6 H  uu_1_specify=off  uu_1_priority=None  uu_1=0 V  uu_1_nominal_specify=off  uu_1_nominal_value=1  uu_1_nominal_unit=V  uv_1_specify=off  uv_1_priority=None  uv_1=0 V  uv_1_nominal_specify=off  uv_1_nominal_value=1  uv_1_nominal_unit=V  uw_1_specify=off  uw_1_priority=None  uw_1=0 V  uw_1_nominal_specify=off  uw_1_nominal_value=1  uw_1_nominal_unit=V  uu_2_specify=off  uu_2_priority=None  uu_2=0 V  uu_2_nominal_specify=off  uu_2_nominal_value=1  uu_2_nominal_unit=V  uv_2_specify=off  uv_2_priority=None  uv_2=0 V  uv_2_nominal_specify=off  uv_2_nominal_value=1  uv_2_nominal_unit=V  uw_2_specify=off  uw_2_priority=None  uw_2=0 V  uw_2_nominal_specify=off  uw_2_nominal_value=1  uw_2_nominal_unit=V  iu_specify=off  iu_priority=High  iu=0 A  iu_nominal_specify=off  iu_nominal_value=1  iu_nominal_unit=A  iv_specify=off  iv_priority=High  iv=0 A  iv_nominal_specify=off  iv_nominal_value=1  iv_nominal_unit=A  iw_specify=off  iw_priority=High  iw=0 A  iw_nominal_specify=off  iw_nominal_value=1  iw_nominal_unit=A
  threephase_vi_measures_stack : Subsystem
  threephase_vi_measures_stack1 : Subsystem
  us_a : PMIOPort  Side=Left
  ug_a : PMIOPort  Port=2  Side=Right
  us_b : PMIOPort  Port=3  Side=Left
  ug_b : PMIOPort  Port=4  Side=Right
  us_c : PMIOPort  Port=5  Side=Left
  ug_c : PMIOPort  Port=6  Side=Right
  connections:
  Inductor2/RConn1 -- threephase_vi_measures_stack1/LConn3 -- CapacitorFilter/LConn3
  Inductor1/RConn1 -- CapacitorFilter/LConn2 -- threephase_vi_measures_stack1/LConn2
  threephase_vi_measures_stack/LConn1 -- us_a/RConn1
  threephase_vi_measures_stack/LConn2 -- us_b/RConn1
  threephase_vi_measures_stack/LConn3 -- us_c/RConn1
  threephase_vi_measures_stack/RConn1 -- threephase inductor/LConn1
  threephase_vi_measures_stack/RConn2 -- threephase inductor/LConn2
  threephase_vi_measures_stack/RConn3 -- threephase inductor/LConn3
  threephase inductor/RConn1 -- Inductor/LConn1
  Inductor1/LConn1 -- threephase inductor/RConn2
  Inductor2/LConn1 -- threephase inductor/RConn3
  ug_a/RConn1 -- threephase_vi_measures_stack1/RConn1
  ug_b/RConn1 -- threephase_vi_measures_stack1/RConn2
  ug_c/RConn1 -- threephase_vi_measures_stack1/RConn3
  threephase_vi_measures_stack1/LConn1 -- CapacitorFilter/LConn1 -- Inductor/RConn1

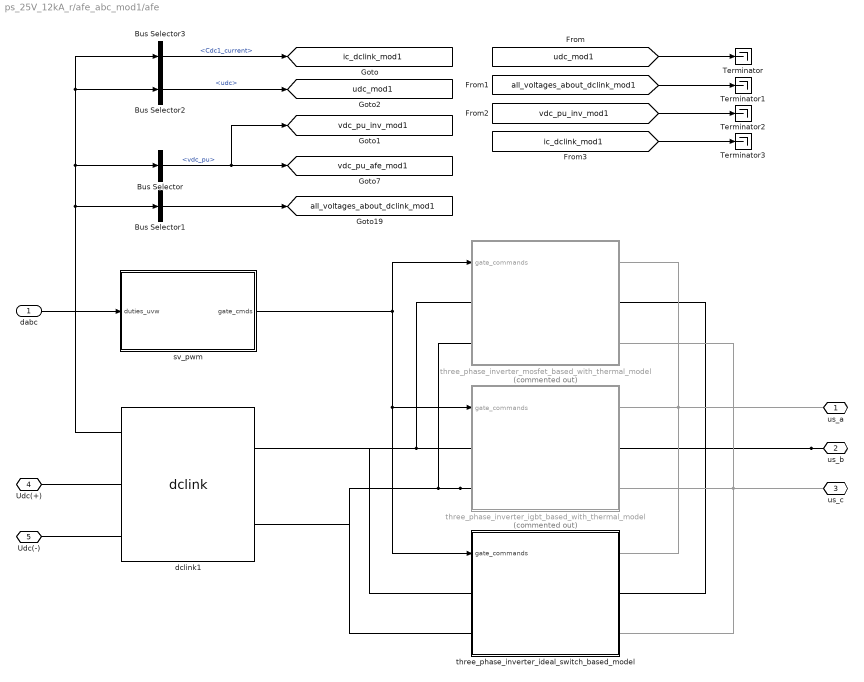
== system ps_25V_12kA_r/afe_abc_mod1/afe ==
  dabc : Inport
  Bus Selector : BusSelector  OutputSignals=vdc_pu
  Bus Selector1 : BusSelector  OutputSignals=udc,udc_p_gnd,udc_centertap_gnd,udc_n_gnd  OutputAsBus=on
  Bus Selector2 : BusSelector  OutputSignals=udc
  Bus Selector3 : BusSelector  OutputSignals=Cdc1_current
  Terminator{,1..3} (4 alike) : Terminator
  dclink1 : dclink_for_two_levels/dclink  Cdc=param.afe.hw.CFi  Rudc_measure=1e6  Vdc_scale=param.afe.hw.udc_nom
  sv_pwm : Subsystem
  three_phase_inverter_ideal_switch_based_model : Subsystem
  three_phase_inverter_igbt_based_with_thermal_model : Subsystem  Commented=on
  three_phase_inverter_mosfet_based_with_thermal_model : Subsystem  Commented=on
  us_a : PMIOPort  Side=Left
  us_b : PMIOPort  Port=2  Side=Left
  us_c : PMIOPort  Port=3  Side=Left
  Udc(+) : PMIOPort  Port=4  Side=Right
  Udc(-) : PMIOPort  Port=5  Side=Right
  tag scope: all_voltages_about_dclink_mod1=global, ic_dclink_mod1=global, udc_mod1=global, vdc_pu_afe_mod1=global, vdc_pu_inv_mod1=global
  wires:
  dabc/1 -> sv_pwm/1(duties_uvw)
  sv_pwm/1(gate_cmds) -> three_phase_inverter_mosfet_based_with_thermal_model/1(gate_commands), three_phase_inverter_ideal_switch_based_model/1(gate_commands), three_phase_inverter_igbt_based_with_thermal_model/1(gate_commands)
  dclink1/1 -> Bus Selector1/1, Bus Selector2/1, Bus Selector3/1, Bus Selector/1
  Bus Selector1/1 -> [all_voltages_about_dclink_mod1]
  Bus Selector/1 -> [vdc_pu_afe_mod1], [vdc_pu_inv_mod1]  "<vdc_pu>"
  Bus Selector2/1 -> [udc_mod1]  "<udc>"
  Bus Selector3/1 -> [ic_dclink_mod1]  "<Cdc1_current>"
  [vdc_pu_inv_mod1] -> Terminator2/1
  [ic_dclink_mod1] -> Terminator3/1
  [all_voltages_about_dclink_mod1] -> Terminator1/1
  [udc_mod1] -> Terminator/1
  connections:
  us_b/RConn1 -- three_phase_inverter_ideal_switch_based_model/RConn2 -- three_phase_inverter_mosfet_based_with_thermal_model/RConn2 -- three_phase_inverter_igbt_based_with_thermal_model/RConn2
  dclink1/RConn1 -- Udc(+)/RConn1
  dclink1/RConn2 -- Udc(-)/RConn1
  three_phase_inverter_igbt_based_with_thermal_model/RConn1 -- three_phase_inverter_ideal_switch_based_model/RConn1 -- three_phase_inverter_mosfet_based_with_thermal_model/RConn1 -- us_a/RConn1
  three_phase_inverter_igbt_based_with_thermal_model/LConn2 -- three_phase_inverter_ideal_switch_based_model/LConn2 -- dclink1/LConn2 -- three_phase_inverter_mosfet_based_with_thermal_model/LConn2
  three_phase_inverter_ideal_switch_based_model/LConn1 -- dclink1/LConn1 -- three_phase_inverter_igbt_based_with_thermal_model/LConn1 -- three_phase_inverter_mosfet_based_with_thermal_model/LConn1
  three_phase_inverter_mosfet_based_with_thermal_model/RConn3 -- three_phase_inverter_ideal_switch_based_model/RConn3 -- us_c/RConn1 -- three_phase_inverter_igbt_based_with_thermal_model/RConn3

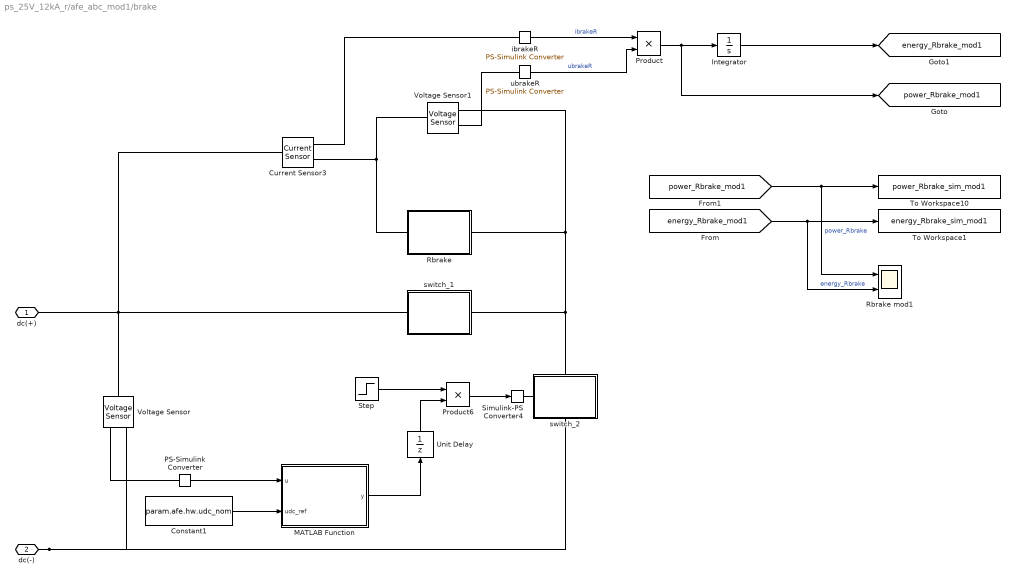
== system ps_25V_12kA_r/afe_abc_mod1/brake ==
  Constant1 : Constant  Value=param.afe.hw.udc_nom
  Current Sensor3 : fl_lib/Electrical/Electrical Sensors/Current Sensor
  Integrator : Integrator
  MATLAB Function : MATLAB Function  TreatAsAtomicUnit=on  SystemSampleTime=param.glb_time.ts_afe
  PS-Simulink Converter : nesl_utility/PS-Simulink Converter  PhysicalDomain=network_engine_domain  SubClassName=ps_output  LeftPortType=input  RightPortType=output  PseudoPeriodic=off  Frequencies=[]  VectorFormat=1-D array  Unit=V  AffineConversion=off
  Product : Product
  Product6 : Product
  Rbrake : Subsystem
  Rbrake mod1 : Scope  NumInputPorts=2
      settings: SampleTime=param.glb_time.tc  ActiveDisplayYMinimum=-85981.043284885527  ActiveDisplayYMaximum=773829.38956396992  DataLoggingVariableName=ScopeData2
  Simulink-PS Converter4 : nesl_utility/Simulink-PS Converter  PhysicalDomain=network_engine_domain  SubClassName=ps_input  LeftPortType=input  RightPortType=output  PseudoPeriodic=off  Frequencies=[]  NoiseDistribution=none  NoiseParameters=[]  Unit=1  AffineConversion=on  FilteringAndDerivatives=provide  SimscapeFilterOrder=1  InputFilterTimeConstant=0.001  UdotUserProvided=0
  Step : Step  Time=param.afe.behav.time_aux_power_supply_fault  InitialValue=1  FinalValue=0  SampleTime=0
  To Workspace1 : ToWorkspace  VariableName=energy_Rbrake_sim_mod1  SampleTime=param.glb_time.tc
      settings: MaxDataPoints=param.glb_time.Nc
  To Workspace10 : ToWorkspace  VariableName=power_Rbrake_sim_mod1  SampleTime=param.glb_time.tc
      settings: MaxDataPoints=param.glb_time.Nc
  Unit Delay : UnitDelay  SampleTime=param.glb_time.ts_afe
  Voltage Sensor : fl_lib/Electrical/Electrical Sensors/Voltage Sensor
  Voltage Sensor1 : fl_lib/Electrical/Electrical Sensors/Voltage Sensor
  ibrakeR : nesl_utility/PS-Simulink Converter  PhysicalDomain=network_engine_domain  SubClassName=ps_output  LeftPortType=input  RightPortType=output  PseudoPeriodic=off  Frequencies=[]  VectorFormat=1-D array  Unit=A  AffineConversion=off
  switch_1 : Subsystem
      settings: PortSchema="{\"entries\":[{\"content\":{\"sides\":[{\"content\":{},\"type\":\"ConnectorPlacement.EquallySpacedRectSide\",\"uuid\":\"9277da8d-d460-43e6-8478-dd662f15d226\"},{\"content\":{\"side\":\"RIGHT\"},\"type\":\"ConnectorPlacement.EquallySpacedRectSide\",\"uuid\":\"a7ece396-f1d9-4f4f-a05b-db1fc65d6e1d\"},{\"content\":{\"connectorIds\":[\"LConn1\"],\"side\":\"TOP\"},\"type\":\"ConnectorPlacement.EquallySpacedRectSide\",\"uuid\":\"fdd70777-e9cf-4317-afb6-cae87f75d5b0\"},{\"content\":{\"connectorIds\":[\"RConn1\"],\"side\":\"BOTTOM\"},\"type\":\"ConnectorPlacement.EquallySpacedRectSide\",\"uuid\":\"2353ed68-b1a1-4775-9ca9-31e268d5443b\"}]},\"type\":\"ConnectorPlacement.EquallySpacedConnector\",\"uuid\":\"d5479f4c-4e65-4791-adcb-73df11f88590\"}],\"packageUris\":[\"http://schema.mathworks.com/mf0/Connector/R2020b\"],\"version\":\"1.0\"}"
  switch_2 : Subsystem
      settings: PortSchema="{\"entries\":[{\"content\":{\"sides\":[{\"content\":{\"connectorIds\":[\"LConn1\"]},\"type\":\"ConnectorPlacement.EquallySpacedRectSide\",\"uuid\":\"9277da8d-d460-43e6-8478-dd662f15d226\"},{\"content\":{\"connectorIds\":[],\"side\":\"RIGHT\"},\"type\":\"ConnectorPlacement.EquallySpacedRectSide\",\"uuid\":\"a7ece396-f1d9-4f4f-a05b-db1fc65d6e1d\"},{\"content\":{\"connectorIds\":[\"LConn2\"],\"side\":\"TOP\"},\"type\":\"ConnectorPlacement.EquallySpacedRectSide\",\"uuid\":\"fdd70777-e9cf-4317-afb6-cae87f75d5b0\"},{\"content\":{\"connectorIds\":[\"RConn1\"],\"side\":\"BOTTOM\"},\"type\":\"ConnectorPlacement.EquallySpacedRectSide\",\"uuid\":\"2353ed68-b1a1-4775-9ca9-31e268d5443b\"}]},\"type\":\"ConnectorPlacement.EquallySpacedConnector\",\"uuid\":\"d5479f4c-4e65-4791-adcb-73df11f88590\"}],\"packageUris\":[\"http://schema.mathworks.com/mf0/Connector/R2020b\"],\"version\":\"1.0\"}"
  ubrakeR : nesl_utility/PS-Simulink Converter  PhysicalDomain=network_engine_domain  SubClassName=ps_output  LeftPortType=input  RightPortType=output  PseudoPeriodic=off  Frequencies=[]  VectorFormat=1-D array  Unit=V  AffineConversion=off
  dc(+) : PMIOPort  Side=Left
  dc(-) : PMIOPort  Port=2  Side=Left
  tag scope: energy_Rbrake_mod1=global, power_Rbrake_mod1=global
  wires:
  Constant1/1 -> MATLAB Function/2(udc_ref)
  PS-Simulink Converter/1 -> MATLAB Function/1(u)
  MATLAB Function/1(y) -> Unit Delay/1
  ibrakeR/1 -> Product/1  "ibrakeR"
  ubrakeR/1 -> Product/2  "ubrakeR"
  Product/1 -> [power_Rbrake_mod1], Integrator/1
  Integrator/1 -> [energy_Rbrake_mod1]
  [power_Rbrake_mod1] -> To Workspace10/1, Rbrake mod1/1  "power_Rbrake"
  [energy_Rbrake_mod1] -> To Workspace1/1, Rbrake mod1/2  "energy_Rbrake"
  Step/1 -> Product6/1
  Unit Delay/1 -> Product6/2
  Product6/1 -> Simulink-PS Converter4/1
  connections:
  dc(-)/RConn1 -- switch_2/RConn1 -- Voltage Sensor/RConn2
  Voltage Sensor1/RConn2 -- Rbrake/RConn1 -- switch_1/RConn1 -- switch_2/LConn2
  PS-Simulink Converter/LConn1 -- Voltage Sensor/RConn1
  switch_2/LConn1 -- Simulink-PS Converter4/RConn1
  Voltage Sensor/LConn1 -- Current Sensor3/LConn1 -- switch_1/LConn1 -- dc(+)/RConn1
  Current Sensor3/RConn1 -- ibrakeR/LConn1
  Voltage Sensor1/RConn1 -- ubrakeR/LConn1
  Current Sensor3/RConn2 -- Voltage Sensor1/LConn1 -- Rbrake/LConn1

== system ps_25V_12kA_r/battery_1/single_phase_ui_measure ==
  Bus Creator : BusCreator  Inputs=2
  Current Sensor : fl_lib/Electrical/Electrical Sensors/Current Sensor
  Selector : Selector  InputPortWidth=2  IndexOptions=Index vector (dialog)  Indices=2  OutputSizes=1  RuntimeRangeChecks=off
  Selector1 : Selector  InputPortWidth=2  IndexOptions=Index vector (dialog)  Indices=1  OutputSizes=1  RuntimeRangeChecks=off
  Terminator : Terminator
  Terminator1 : Terminator
  Voltage Sensor : fl_lib/Electrical/Electrical Sensors/Voltage Sensor
  dab input modA : Scope  NumInputPorts=2
      settings: SampleTime=param.glb_time.tc  ActiveDisplayYMinimum=647.40760725063581  ActiveDisplayYMaximum=862.97823080607691  DataLoggingVariableName=ScopeData2
  iph : nesl_utility/PS-Simulink Converter  PhysicalDomain=network_engine_domain  SubClassName=ps_output  LeftPortType=input  RightPortType=output  PseudoPeriodic=off  Frequencies=[]  VectorFormat=1-D array  Unit=A  AffineConversion=off
  uph : nesl_utility/PS-Simulink Converter  PhysicalDomain=network_engine_domain  SubClassName=ps_output  LeftPortType=input  RightPortType=output  PseudoPeriodic=off  Frequencies=[]  VectorFormat=1-D array  Unit=V  AffineConversion=off
  Udc(+) : PMIOPort  Side=Left
  udc(+) : PMIOPort  Port=2  Side=Right
  Udc(-) : PMIOPort  Port=3  Side=Left
  udc(-) : PMIOPort  Port=4  Side=Right
  tag scope: current_battery_1=global, voltage_battery_1=global
  wires:
  Bus Creator/1 -> Selector/1, Selector1/1  "ui_data"
  iph/1 -> Bus Creator/1  "iph"
  uph/1 -> Bus Creator/2  "uph"
  Selector1/1 -> [current_battery_1], dab input modA/1  "current_battery"
  Selector/1 -> dab input modA/2, [voltage_battery_1]  "voltage_battery"
  [current_battery_1] -> Terminator/1
  [voltage_battery_1] -> Terminator1/1
  connections:
  iph/LConn1 -- Current Sensor/RConn1
  Voltage Sensor/LConn1 -- Current Sensor/LConn1 -- Udc(+)/RConn1
  Current Sensor/RConn2 -- udc(+)/RConn1
  Voltage Sensor/RConn1 -- uph/LConn1
  Voltage Sensor/RConn2 -- Udc(-)/RConn1 -- udc(-)/RConn1

== system ps_25V_12kA_r/full_bridge_converter/full_bridge_converter_with_iso ==
  gate_cmds : Inport
  Bus Selector : BusSelector  OutputSignals=gate_cmd_Q1,gate_cmd_Q2,gate_cmd_Q3,gate_cmd_Q4  OutputAsBus=on
  CFi_dc1 : fl_lib/Electrical/Electrical Elements/Capacitor  c=param.psfbc.hw.Cdc_dc1 F  r=param.psfbc.hw.RCdc_dc1 Ohm  g=0 1/Ohm  i_specify=off  i_priority=None  i=0 A  i_nominal_specify=off  i_nominal_value=1  i_nominal_unit=A  v_specify=off  v_priority=None  v=0 V  v_nominal_specify=off  v_nominal_value=1  v_nominal_unit=V  vc_specify=off  vc_priority=High  vc=0 V  vc_nominal_specify=off  vc_nominal_value=1  vc_nominal_unit=V
  Current Sensor2 : fl_lib/Electrical/Electrical Sensors/Current Sensor
  Current Sensor4 : fl_lib/Electrical/Electrical Sensors/Current Sensor
  PS-Simulink Converter1 : nesl_utility/PS-Simulink Converter  PhysicalDomain=network_engine_domain  SubClassName=ps_output  LeftPortType=input  RightPortType=output  PseudoPeriodic=off  Frequencies=[]  VectorFormat=1-D array  Unit=A  AffineConversion=on
  PS-Simulink Converter6 : nesl_utility/PS-Simulink Converter  PhysicalDomain=network_engine_domain  SubClassName=ps_output  LeftPortType=input  RightPortType=output  PseudoPeriodic=off  Frequencies=[]  VectorFormat=1-D array  Unit=A  AffineConversion=on
  Voltage Sensor2 : fl_lib/Electrical/Electrical Sensors/Voltage Sensor
  full_bridge : Subsystem
      settings: PortSchema="{\"entries\":[{\"content\":{\"sides\":[{\"content\":{\"connectorIds\":[\"LConn1\",\"LConn2\"]},\"type\":\"ConnectorPlacement.EquallySpacedRectSide\",\"uuid\":\"c872503a-61af-4937-bdf2-4de4f8645573\"},{\"content\":{\"connectorIds\":[\"RConn1\",\"RConn2\"],\"side\":\"RIGHT\"},\"type\":\"ConnectorPlacement.EquallySpacedRectSide\",\"uuid\":\"3b83f060-86a2-4569-84b5-d9f7c0485347\"},{\"content\":{\"connectorIds\":[\"In1\"],\"side\":\"TOP\"},\"type\":\"ConnectorPlacement.EquallySpacedRectSide\",\"uuid\":\"bf191d46-ce71-4d15-9dd0-24cc57253577\"}]},\"type\":\"ConnectorPlacement.EquallySpacedConnector\",\"uuid\":\"1b28ceee-25d0-45ae-a3c4-c2563f0d63ba\"}],\"packageUris\":[\"http://schema.mathworks.com/mf0/Connector/R2020b\"],\"version\":\"1.0\"}"
  scopes : Subsystem
  trafo_rectifier : Subsystem
  udc1 : nesl_utility/PS-Simulink Converter  PhysicalDomain=network_engine_domain  SubClassName=ps_output  LeftPortType=input  RightPortType=output  PseudoPeriodic=off  Frequencies=[]  VectorFormat=1-D array  Unit=V  AffineConversion=off
  Udc(+) : PMIOPort  Side=Left
  Udc(-) : PMIOPort  Port=2  Side=Left
  udc_load(+) : PMIOPort  Port=3  Side=Right
  udc_load(-) : PMIOPort  Port=4  Side=Right
  tag scope: CFi_dc1_current=global, psfbc_current_input=global, psfbc_voltage_input=global
  wires:
  gate_cmds/1 -> Bus Selector/1
  PS-Simulink Converter6/1 -> [psfbc_current_input]  "idc"
  Bus Selector/1 -> full_bridge/1(gate_commands)
  udc1/1 -> [psfbc_voltage_input]
  PS-Simulink Converter1/1 -> [CFi_dc1_current]  "CFi_dc1_current"
  connections:
  full_bridge/RConn2 -- Voltage Sensor2/RConn2 -- Current Sensor4/RConn2 -- Udc(-)/RConn1
  full_bridge/RConn1 -- Voltage Sensor2/LConn1 -- Current Sensor2/RConn2 -- CFi_dc1/LConn1
  Udc(+)/RConn1 -- Current Sensor2/LConn1
  Current Sensor2/RConn1 -- PS-Simulink Converter6/LConn1
  Voltage Sensor2/RConn1 -- udc1/LConn1
  Current Sensor4/LConn1 -- CFi_dc1/RConn1
  Current Sensor4/RConn1 -- PS-Simulink Converter1/LConn1
  full_bridge/LConn1 -- trafo_rectifier/LConn1
  trafo_rectifier/RConn1 -- udc_load(+)/RConn1
  full_bridge/LConn2 -- trafo_rectifier/LConn2
  trafo_rectifier/RConn2 -- udc_load(-)/RConn1

== system ps_25V_12kA_r/full_bridge_converter/phase_shift_full_bridge_ctrl ==
  full_bridge_zvs_pwm_modulator : full_bridge_zvs_pwm_modulator/full_bridge_zvs_pwm_modulator  fPWM_m=param.glb_time.fPWM_PSFBC  m_up_m=1  m_low_m=0  dead_time_DAB_m=param.glb_time.dead_time_PSFBC  pos_cmd_gate_m=15  neg_cmd_gate_m=-10  polarity_m=1  tc_m=param.glb_time.tc  max_phase_displacement_m=pi  trgo_double_update_m=param.glb_time.TRGO_PSFBC_double_update
  references : Subsystem
  sampling_i_filter1 : Subsystem
  sampling_i_filter2 : Subsystem
  sampling_v_filter1 : Subsystem
  sampling_v_filter2 : Subsystem
  ui_ctrl : Subsystem
  gate_cmds : Outport
  tag scope: TRGO_PSFBC_1=global, d1m_psfbc=global, phase_disp_psfbc=global
  wires:
  [psfbc_voltage_output] -> sampling_v_filter1/1(in)
  [psfbc_current_output] -> sampling_i_filter1/1(in)
  sampling_i_filter1/1(out_pu) -> ui_ctrl/1(i_pu_dab_input)
  sampling_v_filter1/1(out_pu) -> ui_ctrl/2(u_pu_dab_output)
  sampling_v_filter2/1(out_pu) -> ui_ctrl/3(i_pu_dab_output_ref)
  references/1(vout_ref) -> sampling_v_filter2/1(in)
  full_bridge_zvs_pwm_modulator/2 -> gate_cmds/1
  [time_psfbc_module_1] -> full_bridge_zvs_pwm_modulator/1
  full_bridge_zvs_pwm_modulator/1 -> [TRGO_PSFBC_1]
  [TRGO_PSFBC_1] -> ui_ctrl/Trigger
  [psfbc_current_input] -> sampling_i_filter2/1(in)
  sampling_i_filter2/1(out_pu) -> ui_ctrl/4(i_ac_pu_1)
  ui_ctrl/1(d1m) -> [d1m_psfbc]
  ui_ctrl/2(phase_displacement) -> [phase_disp_psfbc]
  [phase_disp_psfbc] -> full_bridge_zvs_pwm_modulator/3
  [d1m_psfbc] -> full_bridge_zvs_pwm_modulator/2

== system ps_25V_12kA_r/global timing/time_afe1 ==
  correction_time : Inport
  Constant : Constant
  Gain : Gain  Gain=k
  Product : Product
  Sum : Sum  Inputs=|++
  time_1 : Clock
  Out1 : Outport
  wires:
  time_1/1 -> Gain/1
  Gain/1 -> Product/1
  Product/1 -> Out1/1
  correction_time/1 -> Sum/1
  Sum/1 -> Product/2
  Constant/1 -> Sum/2

== system ps_25V_12kA_r/global timing/time_fbc1 ==
  correction_time : Inport
  Constant : Constant
  Gain : Gain  Gain=k
  Product : Product
  Sum : Sum  Inputs=|++
  time_1 : Clock
  Out1 : Outport
  wires:
  Sum/1 -> Product/2
  Constant/1 -> Sum/2
  correction_time/1 -> Sum/1
  Product/1 -> Out1/1
  Gain/1 -> Product/1
  time_1/1 -> Gain/1

== system ps_25V_12kA_r/global timing/time_master ==
  Gain : Gain  Gain=k
  time_1 : Clock
  Out1 : Outport
  wires:
  Gain/1 -> Out1/1
  time_1/1 -> Gain/1
